simulink model "s_b16a4x512f"  (R2016b)
settings: Solver=VariableStepDiscrete  StartTime=0.0  StopTime=1  RelTol=1e-3
undefined symbols (not defined in the file): fft_stages, n_bits_ants, n_bits_xengs
libraries: xbsIndex_r4 x23057, casper_library_misc x150, xbsReplacements_r4 x9, casper_library_delays x8, xps_library x3
(part 59 of 210)

== system s_b16a4x512f/sys2/pack_out_skarab/pack_xeng ==
  note: eof ON the last valid data.
  note: SPEAD header
  note: magic number - 0x53
  note: spead version
  note: item id width in bytes
  note: heap addr width in bytes
  note: <reserved>
  note: num item pointers -
      | after this header
  data256_ready : Inport
  data256_valid : Inport  Port=2
  data256 : Inport  Port=3
  hdr_heap_id : Inport  Port=4
  hdr_heap_size : Inport  Port=5
  hdr_heap_offset : Inport  Port=6
  hdr_pkt_len_words : Inport  Port=7
  hdr5_0x1600_DIR : Inport  Port=8
  hdr6_0x4103_DIR : Inport  Port=9
  hdr8_0x1800 : Inport  Port=10
  AddSub1 : xbsIndex_r4/AddSub  mode=Subtraction  use_carryin=off  use_carryout=off  en=off  latency=0  precision=Full  arith_type=Unsigned  n_bits=16  bin_pt=14  quantization=Truncate  overflow=Wrap  use_behavioral_HDL=off  hw_selection=Fabric  pipelined=off  dbl_ovrd=off  block_type=addsub
  Assert17 : xbsIndex_r4/Assert  assert_type=on  type_source=Explicitly  gui_display_data_type=Fixed-point  arith_type=Unsigned  n_bits=64  bin_pt=0  preci_type=Single  exp_width=8  frac_width=24  assert_rate=off  rate_source=Explicitly  period=1  output_port=on  block_type=assert
  Assert18 : xbsIndex_r4/Assert  assert_type=on  type_source=Explicitly  gui_display_data_type=Fixed-point  arith_type=Unsigned  n_bits=256  bin_pt=0  preci_type=Single  exp_width=8  frac_width=24  assert_rate=off  rate_source=Explicitly  period=1  output_port=on  block_type=assert
  Assert5 : xbsIndex_r4/Assert  assert_type=on  type_source=Explicitly  gui_display_data_type=Fixed-point  arith_type=Boolean  n_bits=64  bin_pt=0  preci_type=Single  exp_width=8  frac_width=24  assert_rate=off  rate_source=Explicitly  period=1  output_port=on  block_type=assert
      settings: block_version=10.1.3
  Assert6 : xbsIndex_r4/Assert  assert_type=on  type_source=Explicitly  gui_display_data_type=Fixed-point  arith_type=Unsigned  n_bits=256  bin_pt=0  preci_type=Single  exp_width=8  frac_width=24  assert_rate=off  rate_source=Explicitly  period=1  output_port=on  block_type=assert
      settings: block_version=10.1.3
  Assert7 : xbsIndex_r4/Assert  assert_type=on  type_source=Explicitly  gui_display_data_type=Boolean  arith_type=Boolean  n_bits=64  bin_pt=0  preci_type=Single  exp_width=8  frac_width=24  assert_rate=off  rate_source=Explicitly  period=1  output_port=on  block_type=assert
      settings: block_version=10.1.3
  Concat : xbsIndex_r4/Concat  num_inputs=6  dbl_ovrd=off  block_type=concat
      settings: block_version=10.1.3
  Concat1 : xbsIndex_r4/Concat  num_inputs=4  dbl_ovrd=off  block_type=concat
      settings: block_version=10.1.3
  Concat3 : xbsIndex_r4/Concat  num_inputs=4  dbl_ovrd=off  block_type=concat
      settings: block_version=10.1.3
  Constant3 : xbsIndex_r4/Constant  const=83  gui_display_data_type=Fixed-point  arith_type=Unsigned  n_bits=8  bin_pt=0  preci_type=Single  exp_width=8  frac_width=24  explicit_period=on  period=1  equ=P=C  opselect=C  inp2=PCIN>>17  opr=+  inp1=P  carry=CIN  dbl_ovrd=off  block_type=constant
  Constant4 : xbsIndex_r4/Constant  const=spead_version  gui_display_data_type=Fixed-point  arith_type=Unsigned  n_bits=8  bin_pt=0  preci_type=Single  exp_width=8  frac_width=24  explicit_period=on  period=1  equ=P=C  opselect=C  inp2=PCIN>>17  opr=+  inp1=P  carry=CIN  dbl_ovrd=off  block_type=constant
  Constant7 : xbsIndex_r4/Constant  const=0  gui_display_data_type=Fixed-point  arith_type=Unsigned  n_bits=16  bin_pt=0  preci_type=Single  exp_width=8  frac_width=24  explicit_period=on  period=1  equ=P=C  opselect=C  inp2=PCIN>>17  opr=+  inp1=P  carry=CIN  dbl_ovrd=off  block_type=constant
  Logical5 : xbsIndex_r4/Logical  logical_function=AND  inputs=2  en=off  latency=0  precision=Full  arith_type=Unsigned  n_bits=8  bin_pt=2  align_bp=on  dbl_ovrd=off  block_type=logical
      settings: xl_area=[0, 0, 0, 0, 0, 0, 0]
  Logical6 : xbsIndex_r4/Logical  logical_function=OR  inputs=2  en=off  latency=0  precision=Full  arith_type=Unsigned  n_bits=8  bin_pt=2  align_bp=on  dbl_ovrd=off  block_type=logical
      settings: xl_area=[0, 0, 0, 0, 0, 0, 0]
  Logical7 : xbsIndex_r4/Logical  logical_function=OR  inputs=2  en=off  latency=1  precision=Full  arith_type=Unsigned  n_bits=8  bin_pt=2  align_bp=on  dbl_ovrd=off  block_type=logical
      settings: xl_area=[0, 0, 0, 0, 0, 0, 0]
  Logical8 : xbsIndex_r4/Logical  logical_function=OR  inputs=2  en=off  latency=0  precision=Full  arith_type=Unsigned  n_bits=8  bin_pt=2  align_bp=on  dbl_ovrd=off  block_type=logical
      settings: xl_area=[0, 0, 0, 0, 0, 0, 0]
  Register2 : xbsIndex_r4/Register  init=0  rst=on  en=on  dbl_ovrd=off  block_type=register
  Relational3 : xbsIndex_r4/Relational  mode=a=b  op_type=Bool  en=off  latency=0  dbl_ovrd=off  block_type=relational
      settings: xl_area=[0, 0, 0, 0, 0, 0, 0]  block_version=10.1.3
  assert_data2 : xbsIndex_r4/Assert  assert_type=on  type_source=Explicitly  gui_display_data_type=Fixed-point  arith_type=Unsigned  n_bits=256  bin_pt=0  preci_type=Single  exp_width=8  frac_width=24  assert_rate=off  rate_source=Explicitly  period=1  output_port=on  block_type=assert
  assert_data3 : xbsIndex_r4/Assert  assert_type=on  type_source=Explicitly  gui_display_data_type=Fixed-point  arith_type=Unsigned  n_bits=256  bin_pt=0  preci_type=Single  exp_width=8  frac_width=24  assert_rate=off  rate_source=Explicitly  period=1  output_port=on  block_type=assert
  data_ctr1 : xbsIndex_r4/Counter  cnt_type=Free Running  cnt_to=4  operation=Up  start_count=0  cnt_by_val=1  arith_type=Unsigned  n_bits=max_pkt_len_bits + 1  bin_pt=0  load_pin=off  rst=on  en=on  explicit_period=on  period=1  use_behavioral_HDL=off  implementation=Fabric  use_rpm=on  dbl_ovrd=off  block_type=counter
      settings: xl_area=[0, 0, 0, 0, 0, 0, 0]
  delay_data{6,9..10,13,15,17..18,20} (8 alike) : xbsIndex_r4/Delay  rst=off  infoeditControl=Selection of Reset will increase slice count due to use of real FFs and instead of SRLs  en=off  latency=1  reg_retiming=on  dbl_ovrd=off  block_type=delay
      settings: block_version=11.4
  delay_data12 : xbsIndex_r4/Delay  rst=off  infoeditControl=Selection of Reset will increase slice count due to use of real FFs and instead of SRLs  en=off  latency=2  reg_retiming=on  dbl_ovrd=off  block_type=delay
      settings: infoedit=Hardware notes: A delay line is a chain, each link of which is an SRL16 or SRL32 followed by a flip-flop.  block_version=11.4
  delay_data5 : xbsIndex_r4/Delay  rst=off  infoeditControl=Selection of Reset will increase slice count due to use of real FFs and instead of SRLs  en=off  latency=2  reg_retiming=on  dbl_ovrd=off  block_type=delay
      settings: infoedit=Hardware notes: A delay line is a chain, each link of which is an SRL16 or SRL32 followed by a flip-flop.  block_version=11.4
  delay_data7 : xbsIndex_r4/Delay  rst=off  infoeditControl=Selection of Reset will increase slice count due to use of real FFs and instead of SRLs  en=off  latency=2  reg_retiming=on  dbl_ovrd=off  block_type=delay
      settings: infoedit=Hardware notes: A delay line is a chain, each link of which is an SRL16 or SRL32 followed by a flip-flop.  block_version=11.4
  hdra_{1..6,8} (7 alike) : xbsIndex_r4/Assert  assert_type=on  type_source=Explicitly  gui_display_data_type=Fixed-point  arith_type=Unsigned  n_bits=spead_lsw  bin_pt=0  preci_type=Single  exp_width=8  frac_width=24  assert_rate=off  rate_source=Explicitly  period=1  output_port=on  block_type=assert
  header_4cast4 : xbsIndex_r4/Convert  gui_display_data_type=Fixed-point  arith_type=Unsigned  n_bits=spead_lsw - 5  bin_pt=0  float_type=Single  exp_bits=8  fraction_bits=24  quantization=Truncate  overflow=Wrap  en=off  latency=1  pipeline=on  dbl_ovrd=off  block_type=convert
  header_4cat4 : xbsIndex_r4/Concat  num_inputs=2  dbl_ovrd=off  block_type=concat
  header_4const2 : xbsIndex_r4/Constant  const=0  gui_display_data_type=Fixed-point  arith_type=Unsigned  n_bits=spead_lsw  bin_pt=0  preci_type=Single  exp_width=8  frac_width=24  explicit_period=on  period=1  equ=P=C  opselect=C  inp2=PCIN>>17  opr=+  inp1=P  carry=CIN  dbl_ovrd=off  block_type=constant
  header_4const4 : xbsIndex_r4/Constant  const=0  gui_display_data_type=Fixed-point  arith_type=Unsigned  n_bits=5  bin_pt=0  preci_type=Single  exp_width=8  frac_width=24  explicit_period=on  period=1  equ=P=C  opselect=C  inp2=PCIN>>17  opr=+  inp1=P  carry=CIN  dbl_ovrd=off  block_type=constant
  header_assert{1..6,8} (7 alike) : xbsIndex_r4/Assert  assert_type=on  type_source=Explicitly  gui_display_data_type=Fixed-point  arith_type=Unsigned  n_bits=spead_msw  bin_pt=0  preci_type=Single  exp_width=8  frac_width=24  assert_rate=off  rate_source=Explicitly  period=1  output_port=on  block_type=assert
  header_cat{1..6,8} (7 alike) : xbsIndex_r4/Concat  num_inputs=2  dbl_ovrd=off  block_type=concat
  header_const1 : xbsIndex_r4/Constant  const=32769  gui_display_data_type=Fixed-point  arith_type=Unsigned  n_bits=spead_msw - spead_lsw  bin_pt=0  preci_type=Single  exp_width=8  frac_width=24  explicit_period=off  period=1  equ=P=C  opselect=C  inp2=PCIN>>17  opr=+  inp1=P  carry=CIN  dbl_ovrd=off  block_type=constant
  header_const2 : xbsIndex_r4/Constant  const=32770  gui_display_data_type=Fixed-point  arith_type=Unsigned  n_bits=spead_msw - spead_lsw  bin_pt=0  preci_type=Single  exp_width=8  frac_width=24  explicit_period=off  period=1  equ=P=C  opselect=C  inp2=PCIN>>17  opr=+  inp1=P  carry=CIN  dbl_ovrd=off  block_type=constant
  header_const3 : xbsIndex_r4/Constant  const=32771  gui_display_data_type=Fixed-point  arith_type=Unsigned  n_bits=spead_msw - spead_lsw  bin_pt=0  preci_type=Single  exp_width=8  frac_width=24  explicit_period=off  period=1  equ=P=C  opselect=C  inp2=PCIN>>17  opr=+  inp1=P  carry=CIN  dbl_ovrd=off  block_type=constant
  header_const4 : xbsIndex_r4/Constant  const=32772  gui_display_data_type=Fixed-point  arith_type=Unsigned  n_bits=spead_msw - spead_lsw  bin_pt=0  preci_type=Single  exp_width=8  frac_width=24  explicit_period=off  period=1  equ=P=C  opselect=C  inp2=PCIN>>17  opr=+  inp1=P  carry=CIN  dbl_ovrd=off  block_type=constant
  header_const5 : xbsIndex_r4/Constant  const=38400  gui_display_data_type=Fixed-point  arith_type=Unsigned  n_bits=spead_msw - spead_lsw  bin_pt=0  preci_type=Single  exp_width=8  frac_width=24  explicit_period=off  period=1  equ=P=C  opselect=C  inp2=PCIN>>17  opr=+  inp1=P  carry=CIN  dbl_ovrd=off  block_type=constant
  header_const6 : xbsIndex_r4/Constant  const=49411  gui_display_data_type=Fixed-point  arith_type=Unsigned  n_bits=spead_msw - spead_lsw  bin_pt=0  preci_type=Single  exp_width=8  frac_width=24  explicit_period=off  period=1  equ=P=C  opselect=C  inp2=PCIN>>17  opr=+  inp1=P  carry=CIN  dbl_ovrd=off  block_type=constant
  header_const8 : xbsIndex_r4/Constant  const=6144  gui_display_data_type=Fixed-point  arith_type=Unsigned  n_bits=spead_msw - spead_lsw  bin_pt=0  preci_type=Single  exp_width=8  frac_width=24  explicit_period=off  period=1  equ=P=C  opselect=C  inp2=PCIN>>17  opr=+  inp1=P  carry=CIN  dbl_ovrd=off  block_type=constant
  heap_addr_width : xbsIndex_r4/Constant  const=spead_lsw/8  gui_display_data_type=Fixed-point  arith_type=Unsigned  n_bits=8  bin_pt=0  preci_type=Single  exp_width=8  frac_width=24  explicit_period=on  period=1  equ=P=C  opselect=C  inp2=PCIN>>17  opr=+  inp1=P  carry=CIN  dbl_ovrd=off  block_type=constant
  item_id_width : xbsIndex_r4/Constant  const=(spead_msw-spead_lsw)/8  gui_display_data_type=Fixed-point  arith_type=Unsigned  n_bits=8  bin_pt=0  preci_type=Single  exp_width=8  frac_width=24  explicit_period=on  period=1  equ=P=C  opselect=C  inp2=PCIN>>17  opr=+  inp1=P  carry=CIN  dbl_ovrd=off  block_type=constant
  mainmux1 : xbsIndex_r4/Mux  inputs=2  en=off  latency=1  precision=Full  arith_type="Signed  (2's comp)"  n_bits=8  bin_pt=2  quantization=Truncate  overflow=Wrap  dbl_ovrd=off  block_type=mux
      settings: xl_area=[0, 0, 0, 0, 0, 0, 0]
  mainmux2 : xbsIndex_r4/Mux  inputs=2  en=off  latency=1  precision=Full  arith_type="Signed  (2's comp)"  n_bits=8  bin_pt=2  quantization=Truncate  overflow=Wrap  dbl_ovrd=off  block_type=mux
      settings: xl_area=[0, 0, 0, 0, 0, 0, 0]
  num_item_pts : xbsIndex_r4/Constant  const=7  gui_display_data_type=Fixed-point  arith_type=Unsigned  n_bits=16  bin_pt=0  preci_type=Single  exp_width=8  frac_width=24  explicit_period=on  period=1  equ=P=C  opselect=C  inp2=PCIN>>17  opr=+  inp1=P  carry=CIN  dbl_ovrd=off  block_type=constant
  only_one1 : xbsIndex_r4/Constant  const=1  gui_display_data_type=Fixed-point  arith_type=Unsigned  n_bits=1  bin_pt=0  preci_type=Single  exp_width=8  frac_width=24  explicit_period=on  period=1  equ=P=C  opselect=C  inp2=PCIN>>17  opr=+  inp1=P  carry=CIN  dbl_ovrd=off  block_type=constant
  data_out : Outport
  valid_out : Outport  Port=2
  eof : Outport  Port=3
  data_overflow : Outport  Port=4
  wires:
  [out_data] -> Assert18/1
  [out_valid] -> valid_out/1
  [out_overflow] -> data_overflow/1
  [out_done] -> eof/1
  Logical8/1 -> [out_done]  "out_done"
  delay_data20/1 -> [out_overflow], Logical8/2  "out_overflow"
  delay_data18/1 -> delay_data20/1
  Logical5/1 -> delay_data18/1  "overflow"
  Register2/1 -> Logical5/1  "busy"
  delay_data17/1 -> Logical8/1
  delay_data15/1 -> delay_data17/1
  Relational3/1 -> delay_data15/1, Register2/2  "done"
  AddSub1/1 -> Relational3/2
  only_one1/1 -> AddSub1/2
  [hdr_4] -> AddSub1/1
  data_ctr1/1 -> Relational3/1  "data_ctr"
  [in_data256] -> delay_data12/1
  delay_data12/1 -> delay_data13/1
  delay_data9/1 -> [out_valid]  "out_valid"
  Logical7/1 -> delay_data9/1
  [header1] -> mainmux2/3
  [header0] -> mainmux2/2
  delay_data7/1 -> Logical6/2, mainmux2/1
  mainmux1/1 -> [out_data]  "out_data"
  delay_data13/1 -> mainmux1/2
  mainmux2/1 -> mainmux1/3
  delay_data10/1 -> mainmux1/1
  delay_data6/1 -> Logical6/1
  Logical6/1 -> Logical7/1, data_ctr1/1, delay_data10/1  "wr_hdr"
  [in_ready] -> delay_data6/1, delay_data7/1, Register2/1, Register2/3, Logical5/2  "in_rdy"
  delay_data5/1 -> Logical7/2, data_ctr1/2  "wr_data"
  [in_valid] -> delay_data5/1
  assert_data3/1 -> [header1]
  Concat3/1 -> assert_data3/1
  assert_data2/1 -> [header0]
  Concat1/1 -> assert_data2/1
  header_cat8/1 -> header_assert8/1
  [hdr_8] -> header_cat8/2
  header_const8/1 -> header_cat8/1  "spid8"
  hdra_8/1 -> [hdr_8]  "hdr8_0x4300"
  hdr8_0x1800/1 -> hdra_8/1
  header_assert8/1 -> Concat3/4
  header_assert6/1 -> Concat3/3
  header_cat6/1 -> header_assert6/1
  [hdr_6] -> header_cat6/2
  header_const6/1 -> header_cat6/1  "spid6"
  hdra_6/1 -> [hdr_6]  "hdr6_0x4101_DIR"
  hdr6_0x4103_DIR/1 -> hdra_6/1
  header_assert5/1 -> Concat3/2
  header_cat5/1 -> header_assert5/1
  [hdr_5] -> header_cat5/2
  header_const5/1 -> header_cat5/1  "spid5"
  hdra_5/1 -> [hdr_5]  "hdr5_0x1600_DIR"
  hdr5_0x1600_DIR/1 -> hdra_5/1
  header_assert4/1 -> Concat3/1
  header_cat4/1 -> header_assert4/1
  header_4cat4/1 -> header_cat4/2
  header_4const4/1 -> header_4cat4/2
  header_4cast4/1 -> header_4cat4/1
  [hdr_4] -> header_4cast4/1
  header_const4/1 -> header_cat4/1  "spid4"
  hdra_4/1 -> [hdr_4]  "hdr_pkt_len_words"
  hdr_pkt_len_words/1 -> hdra_4/1
  header_assert3/1 -> Concat1/4
  header_cat3/1 -> header_assert3/1
  [hdr_3] -> header_cat3/2
  header_const3/1 -> header_cat3/1  "spid3"
  hdra_3/1 -> [hdr_3]  "hdr_heap_offset"
  hdr_heap_offset/1 -> hdra_3/1
  header_assert2/1 -> Concat1/3
  header_cat2/1 -> header_assert2/1
  [hdr_2] -> header_cat2/2
  header_const2/1 -> header_cat2/1  "spid2"
  hdra_2/1 -> [hdr_2]  "hdr_heap_size"
  hdr_heap_size/1 -> hdra_2/1
  header_assert1/1 -> Concat1/2
  header_cat1/1 -> header_assert1/1
  [hdr_1] -> header_cat1/2
  header_const1/1 -> header_cat1/1  "spid1"
  hdra_1/1 -> [hdr_1]  "hdr_heap_id"
  hdr_heap_id/1 -> hdra_1/1
  num_item_pts/1 -> Concat/6
  Assert18/1 -> data_out/1
  Assert17/1 -> Concat1/1
  Assert7/1 -> [in_valid]  "data64_valid"
  data256_valid/1 -> Assert7/1
  data256_ready/1 -> Assert5/1
  Assert5/1 -> [in_ready]  "data64_rdy"
  Assert6/1 -> [in_data256]  "data64"
  data256/1 -> Assert6/1
  Constant7/1 -> Concat/5
  heap_addr_width/1 -> Concat/4
  item_id_width/1 -> Concat/3
  Constant4/1 -> Concat/2
  Constant3/1 -> Concat/1
  Concat/1 -> Assert17/1  "spd_hdr"

== system s_b16a4x512f/sys2/pkt_reord/bus_expand ==
  bus_in : Inport
  reinterpret1 : xbsIndex_r4/Reinterpret  force_arith_type=on  arith_type=Unsigned  force_bin_pt=on  bin_pt=0  block_type=reinterpret
  slice1 : xbsIndex_r4/Slice  nbits=32  boolean_output=off  mode=Upper Bit Location + Width  bit1=-1  base1=MSB of Input  bit0=0  base0=LSB of Input  dbl_ovrd=off  block_type=slice
  slice2 : xbsIndex_r4/Slice  nbits=1  boolean_output=on  mode=Upper Bit Location + Width  bit1=0  base1=MSB of Input  bit0=0  base0=LSB of Input  dbl_ovrd=off  block_type=slice
  msb_out2 : Outport
  lsb_out1 : Outport  Port=2
  wires:
  bus_in/1 -> slice2/1, slice1/1
  slice2/1 -> msb_out2/1
  slice1/1 -> reinterpret1/1
  reinterpret1/1 -> lsb_out1/1

== system s_b16a4x512f/sys2/pkt_reord/bus_replicate ==
  in : Inport
  bussify : Subsystem  AncestorBlock=casper_library_flow_control/bus_create  mask(bus_create){inputNum=1}
      mask prompts: inputNum "Number of inputs:"
      mask init:
      | bus_create_init(gcb,...
      |     'inputNum', inputNum);
  out : Outport
  wires:
  in/1 -> bussify/1(in1)
  bussify/1(bus_out) -> out/1

== system s_b16a4x512f/sys2/pkt_reord/input_control ==
  note: signal discard if timestamp
      | changing i.e new packet
      | and not writing
      | and valid
  note: Allow writing to windows
      | up to 1/2 the total buffer size
      |  behind the current maximum
      | mcnt
  data_in : Inport
  valid : Inport  Port=2
  pkt_idx : Inport  Port=3
  time_freq : Inport  Port=4
  src : Inport  Port=5
  pkt_size : Inport  Port=6
  n_src : Inport  Port=7
  AddSub2 : xbsIndex_r4/AddSub  mode=Addition  use_carryin=off  use_carryout=off  en=off  latency=2  precision=User Defined  arith_type=Unsigned  n_bits=n_bits_timestamp+chan_bits-xeng_bits  bin_pt=0  quantization=Truncate  overflow=Wrap  use_behavioral_HDL=on  hw_selection=Fabric  pipelined=off  use_rpm=on  dbl_ovrd=off  block_type=addsub
      settings: xl_area=[0, 0, 0, 0, 0, 0, 0]  block_version=10.1.3
  Constant2 : xbsIndex_r4/Constant  const=2^(window_bits - 1)  gui_display_data_type=Fixed-point  arith_type=Unsigned  n_bits=n_bits_timestamp+chan_bits-xeng_bits  bin_pt=0  preci_type=Single  exp_width=8  frac_width=24  explicit_period=on  period=1  equ=P=C  opselect=C  inp2=PCIN>>17  opr=+  inp1=P  carry=CIN  dbl_ovrd=off  block_type=constant
  Constant4 : xbsIndex_r4/Constant  const=0  gui_display_data_type=Boolean  arith_type=Boolean  n_bits=16  bin_pt=14  preci_type=Single  exp_width=8  frac_width=24  explicit_period=on  period=1  equ=P=C  opselect=C  inp2=PCIN>>17  opr=+  inp1=P  carry=CIN  dbl_ovrd=off  block_type=constant
      settings: block_version=11.4
  Delay{6,11,13..16} (6 alike) : xbsIndex_r4/Delay  rst=off  infoeditControl=Selection of Reset will increase slice count due to use of real FFs and instead of SRLs  en=off  latency=1  reg_retiming=on  dbl_ovrd=off  block_type=delay
      Delay11 settings: infoedit=Hardware notes: A delay line is a chain, each link of which is an SRL16 or SRL32 followed by a flip-flop.  xl_area=[0, 0, 0, 0, 0, 0, 0]
      Delay13 settings: infoedit=Hardware notes: A delay line is a chain, each link of which is an SRL16 or SRL32 followed by a flip-flop.  xl_area=[0, 0, 0, 0, 0, 0, 0]
      Delay14 settings: infoedit=Hardware notes: A delay line is a chain, each link of which is an SRL16 or SRL32 followed by a flip-flop.  xl_area=[0, 0, 0, 0, 0, 0, 0]
      Delay15 settings: infoedit=Hardware notes: A delay line is a chain, each link of which is an SRL16 or SRL32 followed by a flip-flop.  xl_area=[0, 0, 0, 0, 0, 0, 0]
      Delay16 settings: infoedit=Hardware notes: A delay line is a chain, each link of which is an SRL16 or SRL32 followed by a flip-flop.  xl_area=[0, 0, 0, 0, 0, 0, 0]
      Delay6 settings: xl_area=[0, 0, 0, 0, 0, 0, 0]
  Delay{2,4..5,8..9} (5 alike) : xbsIndex_r4/Delay  rst=off  infoeditControl=Selection of Reset will increase slice count due to use of real FFs and instead of SRLs  en=off  latency=2  reg_retiming=on  dbl_ovrd=off  block_type=delay
      settings: xl_area=[0, 0, 0, 0, 0, 0, 0]
  Delay{3,21,24..27} (6 alike) : xbsIndex_r4/Delay  rst=off  infoeditControl=Selection of Reset will increase slice count due to use of real FFs and instead of SRLs  en=off  latency=3  reg_retiming=on  dbl_ovrd=off  block_type=delay
      settings: xl_area=[0, 0, 0, 0, 0, 0, 0]
  Delay23 : xbsIndex_r4/Delay  rst=off  infoeditControl=Selection of Reset will increase slice count due to use of real FFs and instead of SRLs  en=off  latency=4  reg_retiming=on  dbl_ovrd=off  block_type=delay
      settings: xl_area=[0, 0, 0, 0, 0, 0, 0]
  Gateway Out{1..19} (19 alike) : xbsIndex_r4/Gateway Out  inherit_from_input=off  hdl_port=off  rows=1  columns=1  UseAsDAC=off  DACChannel='1'  interface=None  automatic_assignment=on  address_offset=hex2dec('00')  intf_name=''  intf_description=''  timing_constraint=None  locs_specified=off  LOCs={}  io_standard={}  block_type=gatewayout
      settings: infoedit="Gateway out block.  Converts Xilinx fixed point inputs into ouputs of type Simulink integer, double, or fixed point.<P><P>Hardware notes:  In hardware these blocks become top level output ports or are discarded, depending on how they are configured."  xl_area=[0, 0, 0, 0, 0, 0, 0]  block_version=10.1.3
  Inverter : xbsIndex_r4/Inverter  en=off  latency=0  dbl_ovrd=off  block_type=inv
  Logical : xbsIndex_r4/Logical  logical_function=AND  inputs=3  en=off  latency=1  precision=Full  arith_type=Unsigned  n_bits=8  bin_pt=2  align_bp=on  dbl_ovrd=off  block_type=logical
      settings: xl_area=[0, 0, 0, 0, 0, 0, 0]
  Logical1 : xbsIndex_r4/Logical  logical_function=AND  inputs=3  en=off  latency=0  precision=Full  arith_type=Unsigned  n_bits=8  bin_pt=2  align_bp=on  dbl_ovrd=off  block_type=logical
      settings: xl_area=[0, 0, 0, 0, 0, 0, 0]
  Mult : xbsIndex_r4/Mult  precision=Full  arith_type=Unsigned  n_bits=buf_bits  bin_pt=0  quantization=Truncate  overflow=Wrap  en=off  latency=3  use_behavioral_HDL=off  opt=Speed  use_embedded=on  optimum_pipeline=off  pipeline=on  dbl_ovrd=off  use_rpm=on  placement_style=Triangular  block_type=mult
  Mult1 : xbsIndex_r4/Mult  precision=Full  arith_type=Unsigned  n_bits=buf_bits  bin_pt=0  quantization=Truncate  overflow=Wrap  en=off  latency=3  use_behavioral_HDL=off  opt=Speed  use_embedded=on  optimum_pipeline=off  pipeline=on  dbl_ovrd=off  use_rpm=on  placement_style=Triangular  block_type=mult
  Relational : xbsIndex_r4/Relational  mode=a>=b  op_type=Bool  en=off  latency=2  dbl_ovrd=off  block_type=relational
      settings: xl_area=[0, 0, 0, 0, 0, 0, 0]  block_version=10.1.3
  Relational1 : xbsIndex_r4/Relational  mode=a!=b  op_type=Bool  en=off  latency=2  dbl_ovrd=off  block_type=relational
  Relational2 : xbsIndex_r4/Relational  mode=a<b  op_type=Bool  en=off  latency=2  dbl_ovrd=off  block_type=relational
      settings: xl_area=[0, 0, 0, 0, 0, 0, 0]  block_version=10.1.3
  Scope : Scope  NumInputPorts=7
  Slice1 : xbsIndex_r4/Slice  nbits=buf_bits  boolean_output=off  mode=Lower Bit Location + Width  bit1=0  base1=MSB of Input  bit0=0  base0=LSB of Input  dbl_ovrd=off  block_type=slice
  Slice2 : xbsIndex_r4/Slice  nbits=window_bits  boolean_output=off  mode=Lower Bit Location + Width  bit1=0  base1=MSB of Input  bit0=0  base0=LSB of Input  dbl_ovrd=off  block_type=slice
  Slice5 : xbsIndex_r4/Slice  nbits=8  boolean_output=off  mode=Lower Bit Location + Width  bit1=0  base1=MSB of Input  bit0=0  base0=LSB of Input  dbl_ovrd=off  block_type=slice
  Terminator : Terminator
  adder_tree : Subsystem  AncestorBlock=casper_library_misc/adder_tree  mask(adder_tree){n_inputs=3, latency=2, adder_imp=Fabric, first_stage_hdl=off}
      mask prompts: n_inputs "Number of Inputs"; latency "Add Latency"; adder_imp "Adder implementation"; first_stage_hdl "Use behavioural HDL for first stage of adders"
      mask help:
      | Sums all inputs using a tree of adds and delays.
      |
      | Number of inputs: The number of inputs to the block to be summed
      | Add latency: The number of clock cycles to perform one addition (affects timing)..
      | Adder implementation: choice of fabric or DSP48E core, or behavioral HDL
      | Use behavioural HDL for first stage of adders: Causes the first stage of adders to be absorbed into DSP blocks if multipliers precede them (Virtex 5). Overrides Adder implementation
      mask init:
      | adder_tree_init(gcb, ...
      |     'n_inputs', n_inputs, ...
      |     'latency', latency, ...
      |     'adder_imp', adder_imp, ...
      |     'first_stage_hdl', first_stage_hdl);
      settings: AttributesFormatString=latency 4
      mask Help: eval('xlWeb(''http://casper.berkeley.edu/wiki/Adder_tree'')')
      mask TypeOptions adder_imp: Behavioral | Fabric | DSP48
  freq_window : xbsIndex_r4/Mult  precision=Full  arith_type="Signed  (2's comp)"  n_bits=16  bin_pt=14  quantization=Truncate  overflow=Wrap  en=off  latency=3  use_behavioral_HDL=off  opt=Speed  use_embedded=on  optimum_pipeline=off  pipeline=on  dbl_ovrd=off  use_rpm=on  placement_style=Triangular  block_type=mult
  internal_descr_Scope2 : Scope  NumInputPorts=6
  internal_descr_Scope3 : Scope  NumInputPorts=6
  mcnt_thresh : Subsystem
  maxcnt : Outport
  wr_addr : Outport  Port=2
  wr_data : Outport  Port=3
  we : Outport  Port=4
  discarding : Outport  Port=5
  mcnt_timeout : Outport  Port=6
  wires:
  Constant2/1 -> AddSub2/2
  Delay2/1 -> Delay4/1
  Delay3/1 -> Delay2/1, [data_add]
  data_in/1 -> Delay3/1
  adder_tree/2(dout) -> Slice1/1
  Gateway Out15/1 -> internal_descr_Scope3/6
  [brds_pkt_size_time] -> Gateway Out15/1
  [src_pkt_size] -> Gateway Out9/1
  Slice5/1 -> Gateway Out6/1
  Gateway Out1/1 -> internal_descr_Scope3/2
  Gateway Out6/1 -> internal_descr_Scope3/1
  Gateway Out7/1 -> internal_descr_Scope3/3
  Gateway Out9/1 -> internal_descr_Scope3/4
  Gateway Out14/1 -> internal_descr_Scope3/5
  [data_add] -> Slice5/1
  [valid_add] -> Gateway Out1/1
  [pkt_idx] -> Gateway Out7/1
  [wr_addr] -> Gateway Out14/1
  [wr_data] -> Gateway Out3/1
  Gateway Out2/1 -> internal_descr_Scope2/2
  Gateway Out3/1 -> internal_descr_Scope2/1
  Gateway Out4/1 -> internal_descr_Scope2/3
  Gateway Out5/1 -> internal_descr_Scope2/4
  Gateway Out16/1 -> internal_descr_Scope2/5
  [we] -> Gateway Out2/1
  [mcnt_in] -> Gateway Out4/1
  [max_mcnt] -> Gateway Out5/1
  [wr_addr] -> Gateway Out16/1
  Slice2/1 -> Mult1/2
  freq_window/1 -> Mult1/1
  n_src/1 -> freq_window/1
  Mult1/1 -> adder_tree/2(din1), [brds_pkt_size_time]
  Delay27/1 -> AddSub2/1
  Delay26/1 -> mcnt_thresh/1(mcnt)
  Delay25/1 -> Delay5/1
  Constant4/1 -> adder_tree/1(sync)
  Mult/1 -> adder_tree/3(din2), [src_pkt_size]
  Delay21/1 -> [pkt_idx], adder_tree/4(din3)
  time_freq/1 -> Slice2/1, Delay26/1, Delay25/1, [mcnt_in], Delay27/1
  Delay24/1 -> mcnt_thresh/2(en), [valid_add], Delay23/1
  src/1 -> Mult/1
  pkt_size/1 -> freq_window/2, Mult/2
  pkt_idx/1 -> Delay21/1
  valid/1 -> Delay24/1
  Delay9/1 -> Delay13/1
  Slice1/1 -> Delay16/1
  Delay4/1 -> Delay11/1
  Delay23/1 -> Gateway Out13/1, Logical/3, Delay14/1
  Logical/1 -> [we], Inverter/1, we/1
  Relational/1 -> Gateway Out12/1, Logical/2
  Delay5/1 -> Gateway Out10/1, Relational/2, Relational1/1, Delay6/1
  mcnt_thresh/1(maxcnt) -> Delay9/1, Relational2/1, Relational/1, Gateway Out19/1
  Relational2/1 -> Logical/1, Gateway Out11/1
  adder_tree/1(sync_out) -> Terminator/1
  Logical1/1 -> [discarding], discarding/1
  Inverter/1 -> Logical1/1
  Relational1/1 -> Delay15/1, Gateway Out17/1
  Delay6/1 -> Relational1/2
  mcnt_thresh/2(mcnt_timeout) -> Delay8/1
  [discarding] -> Gateway Out8/1
  Gateway Out8/1 -> internal_descr_Scope2/6
  Gateway Out11/1 -> Scope/4
  Gateway Out18/1 -> Scope/3
  Gateway Out13/1 -> Scope/6
  Gateway Out17/1 -> Scope/7
  Gateway Out12/1 -> Scope/5
  Gateway Out10/1 -> Scope/1
  Gateway Out19/1 -> Scope/2
  AddSub2/1 -> Gateway Out18/1, Relational2/2
  Delay11/1 -> wr_data/1, [wr_data]
  Delay13/1 -> maxcnt/1, [max_mcnt]
  Delay14/1 -> Logical1/2
  Delay15/1 -> Logical1/3
  Delay8/1 -> mcnt_timeout/1
  Delay16/1 -> [wr_addr], wr_addr/1

== system s_b16a4x512f/sys2/pkt_reord/munge ==
  din : Inport
  join : Subsystem  AncestorBlock=casper_library_flow_control/bus_create  mask(bus_create){inputNum=16}
      mask prompts: inputNum "Number of inputs:"
      mask init:
      | bus_create_init(gcb,...
      |     'inputNum', inputNum);
  reinterpret : xbsIndex_r4/Reinterpret  force_arith_type=on  arith_type=Unsigned  force_bin_pt=on  bin_pt=0  block_type=reinterpret
  reinterpret_out : xbsIndex_r4/Reinterpret  force_arith_type=on  arith_type=Unsigned  force_bin_pt=on  bin_pt=0  block_type=reinterpret
  split : Subsystem  AncestorBlock=casper_library_flow_control/bus_expand  mask(bus_expand){mode=divisions of arbitrary size, outputNum=1, outputWidth=[1 32 32 32 32 32 32 32 32], outputBinaryPt=[0 0 0 0 0 0 0 0 0], outputArithmeticType=[0 0 0 0 0 0 0 0 0], show_format=off, outputToWorkspace=off, variablePrefix=out, outputToModelAsWell=on}
      mask prompts: outputNum "Number of outputs:"; outputWidth "Output width [msb ... lsb]:"; outputBinaryPt "Output binary point position [msb ... lsb]:"; outputArithmeticType "Output arithmetic type (ufix=0, fix=1, bool=2) [msb ... lsb]:"; show_format "Print format string?"; outputToWorkspace "Output to workspace?"; variablePrefix "Variable name prefix:"; outputToModelAsWell "Output to model as well?"
      mask help:
      | Expands a 'bus' made using a bus_create or Xilinx
      | concat block.
      | The input will be divided into the specified number
      | of outputs with the specified arithmetic types.
      | Divisions are made from most significant bit.
      mask init: same as s_b16a4x512f/bus_expand
      settings: AttributesFormatString=9 outputs
      mask TypeOptions mode: divisions of equal size | divisions of arbitrary size
      mask Callback mode: bus_expand_callback();
      mask Callback outputWidth: bus_expand_callback();
      mask Callback outputToWorkspace: bus_expand_callback();
  dout : Outport
  wires:
  reinterpret_out/1 -> dout/1
  din/1 -> reinterpret/1
  reinterpret/1 -> split/1(bus_in)
  join/1(bus_out) -> reinterpret_out/1
  split/1(msb_out9) -> join/1(in1), join/3(in3), join/5(in5), join/7(in7), join/9(in9), join/11(in11), join/13(in13), join/15(in15)
  split/9(lsb_out1) -> join/2(in2)
  split/8(out2) -> join/4(in4)
  split/7(out3) -> join/6(in6)
  split/6(out4) -> join/8(in8)
  split/5(out5) -> join/10(in10)
  split/4(out6) -> join/12(in12)
  split/3(out7) -> join/14(in14)
  split/2(out8) -> join/16(in16)

== system s_b16a4x512f/sys2/pkt_reord/munge1 ==
  din : Inport
  join : Subsystem  AncestorBlock=casper_library_flow_control/bus_create  mask(bus_create){inputNum=2}
      mask prompts: inputNum "Number of inputs:"
      mask init:
      | bus_create_init(gcb,...
      |     'inputNum', inputNum);
  reinterpret : xbsIndex_r4/Reinterpret  force_arith_type=on  arith_type=Unsigned  force_bin_pt=on  bin_pt=0  block_type=reinterpret
  reinterpret_out : xbsIndex_r4/Reinterpret  force_arith_type=on  arith_type=Unsigned  force_bin_pt=on  bin_pt=0  block_type=reinterpret
  split : Subsystem  AncestorBlock=casper_library_flow_control/bus_expand  mask(bus_expand){mode=divisions of arbitrary size, outputNum=1, outputWidth=[1 32], outputBinaryPt=[0 0], outputArithmeticType=[0 0], show_format=off, outputToWorkspace=off, variablePrefix=out, outputToModelAsWell=on}
      mask prompts: outputNum "Number of outputs:"; outputWidth "Output width [msb ... lsb]:"; outputBinaryPt "Output binary point position [msb ... lsb]:"; outputArithmeticType "Output arithmetic type (ufix=0, fix=1, bool=2) [msb ... lsb]:"; show_format "Print format string?"; outputToWorkspace "Output to workspace?"; variablePrefix "Variable name prefix:"; outputToModelAsWell "Output to model as well?"
      mask help:
      | Expands a 'bus' made using a bus_create or Xilinx
      | concat block.
      | The input will be divided into the specified number
      | of outputs with the specified arithmetic types.
      | Divisions are made from most significant bit.
      mask init: same as s_b16a4x512f/bus_expand
      settings: AttributesFormatString=2 outputs
      mask TypeOptions mode: divisions of equal size | divisions of arbitrary size
      mask Callback mode: bus_expand_callback();
      mask Callback outputWidth: bus_expand_callback();
      mask Callback outputToWorkspace: bus_expand_callback();
  dout : Outport
  wires:
  reinterpret_out/1 -> dout/1
  din/1 -> reinterpret/1
  reinterpret/1 -> split/1(bus_in)
  join/1(bus_out) -> reinterpret_out/1
  split/1(msb_out2) -> join/1(in1)
  split/2(lsb_out1) -> join/2(in2)

== system s_b16a4x512f/sys2/pkt_reord/output_control ==
  note: add delay here
      | to ensure mcnt has had
      | chance to calculate
      | correctly
  note: If reading from addr 0 (corresponding to f=0,nant,2nant,...)
      | and max_mcnt (skipping window_bits for the difference
      | between max_mcnt and rd_mcnt) is 0 for sync_bits, then
      | issue a sync.
  note: If we need to ship a window,
      | send the data on a window edge
  note: Decide whether to ship
      | a window or not:
  note: If the read window is 1/2
      | the total buffer size (or more)
      | behind the write window,
      | it is time to ship it out.
  note: rd_addr is counting for
      | output words to
      | X engines
  maxcnt : Inport
  AddSub1 : xbsIndex_r4/AddSub  mode=Subtraction  use_carryin=off  use_carryout=off  en=off  latency=2  precision=User Defined  arith_type=Unsigned  n_bits=window_bits  bin_pt=0  quantization=Truncate  overflow=Wrap  use_behavioral_HDL=on  hw_selection=Fabric  pipelined=off  use_rpm=on  dbl_ovrd=off  block_type=addsub
      settings: xl_area=[0, 0, 0, 0, 0, 0, 0]  block_version=10.1.3
  Concat1 : xbsIndex_r4/Concat  num_inputs=2  dbl_ovrd=off  block_type=concat
      settings: block_version=10.1.3
  Concat2 : xbsIndex_r4/Concat  num_inputs=2  dbl_ovrd=off  block_type=concat
      settings: block_version=10.1.3
  Constant1 : xbsIndex_r4/Constant  const=2^(window_bits - 1)  gui_display_data_type=Fixed-point  arith_type=Unsigned  n_bits=window_bits  bin_pt=0  preci_type=Single  exp_width=8  frac_width=24  explicit_period=on  period=1  equ=P=C  opselect=C  inp2=PCIN>>17  opr=+  inp1=P  carry=CIN  dbl_ovrd=off  block_type=constant
  Constant3 : xbsIndex_r4/Constant  const=0  gui_display_data_type=Fixed-point  arith_type=Unsigned  n_bits=sync_bits - x_int_bits - ant_bits - window_bits  bin_pt=0  preci_type=Single  exp_width=8  frac_width=24  explicit_period=on  period=1  equ=P=C  opselect=C  inp2=PCIN>>17  opr=+  inp1=P  carry=CIN  dbl_ovrd=off  block_type=constant
  Delay1 : xbsIndex_r4/Delay  rst=off  infoeditControl=Selection of Reset will increase slice count due to use of real FFs and instead of SRLs  en=off  latency=1  reg_retiming=on  dbl_ovrd=off  block_type=delay
      settings: xl_area=[0, 0, 0, 0, 0, 0, 0]
  Delay3 : xbsIndex_r4/Delay  rst=off  infoeditControl=Selection of Reset will increase slice count due to use of real FFs and instead of SRLs  en=off  latency=2  reg_retiming=on  dbl_ovrd=off  block_type=delay
      settings: xl_area=[0, 0, 0, 0, 0, 0, 0]
  Delay6 : xbsIndex_r4/Delay  rst=off  infoeditControl=Selection of Reset will increase slice count due to use of real FFs and instead of SRLs  en=off  latency=1  reg_retiming=on  dbl_ovrd=off  block_type=delay
      settings: xl_area=[0, 0, 0, 0, 0, 0, 0]
  Delay7 : xbsIndex_r4/Delay  rst=off  infoeditControl=Selection of Reset will increase slice count due to use of real FFs and instead of SRLs  en=off  latency=2  reg_retiming=on  dbl_ovrd=off  block_type=delay
      settings: xl_area=[0, 0, 0, 0, 0, 0, 0]
  Gateway Out{1..18} (18 alike) : xbsIndex_r4/Gateway Out  inherit_from_input=off  hdl_port=off  rows=1  columns=1  UseAsDAC=off  DACChannel='1'  interface=None  automatic_assignment=on  address_offset=hex2dec('00')  intf_name=''  intf_description=''  timing_constraint=None  locs_specified=off  LOCs={}  io_standard={}  block_type=gatewayout
      settings: infoedit="Gateway out block.  Converts Xilinx fixed point inputs into ouputs of type Simulink integer, double, or fixed point.<P><P>Hardware notes:  In hardware these blocks become top level output ports or are discarded, depending on how they are configured."  xl_area=[0, 0, 0, 0, 0, 0, 0]  block_version=10.1.3
  Logical1 : xbsIndex_r4/Logical  logical_function=AND  inputs=2  en=off  latency=0  precision=Full  arith_type=Unsigned  n_bits=8  bin_pt=2  align_bp=on  dbl_ovrd=off  block_type=logical
      settings: xl_area=[0, 0, 0, 0, 0, 0, 0]
  Logical2 : xbsIndex_r4/Logical  logical_function=AND  inputs=2  en=off  latency=0  precision=Full  arith_type=Unsigned  n_bits=8  bin_pt=2  align_bp=on  dbl_ovrd=off  block_type=logical
      settings: xl_area=[0, 0, 0, 0, 0, 0, 0]
  Logical4 : xbsIndex_r4/Logical  logical_function=AND  inputs=2  en=off  latency=0  precision=Full  arith_type=Unsigned  n_bits=8  bin_pt=2  align_bp=on  dbl_ovrd=off  block_type=logical
      settings: xl_area=[0, 0, 0, 0, 0, 0, 0]
  Register : xbsIndex_r4/Register  init=0  rst=off  en=on  dbl_ovrd=off  block_type=register
  Register1 : xbsIndex_r4/Register  init=0  rst=off  en=on  dbl_ovrd=off  block_type=register
  Register3 : xbsIndex_r4/Register  init=0  rst=off  en=on  dbl_ovrd=off  block_type=register
  Relational1 : xbsIndex_r4/Relational  mode=a>=b  op_type=Bool  en=off  latency=1  dbl_ovrd=off  block_type=relational
      settings: xl_area=[0, 0, 0, 0, 0, 0, 0]  block_version=10.1.3
  Relational4 : xbsIndex_r4/Relational  mode=a=b  op_type=Bool  en=off  latency=1  dbl_ovrd=off  block_type=relational
      settings: xl_area=[0, 0, 0, 0, 0, 0, 0]  block_version=10.1.3
  Slice1 : xbsIndex_r4/Slice  nbits=window_bits  boolean_output=off  mode=Lower Bit Location + Width  bit1=0  base1=MSB of Input  bit0=0  base0=LSB of Input  dbl_ovrd=off  block_type=slice
      settings: infoedit="Extracts a given range of bits from each input sample and presents it at the output.  The output type is ordinarily unsigned with binary point at zero, but can be Boolean when the slice is one bit wide.<P><P>Hardware notes: In hardware this block costs nothing."  block_version=10.1.3
  Slice2 : xbsIndex_r4/Slice  nbits=1  boolean_output=on  mode=Upper Bit Location + Width  bit1=0  base1=MSB of Input  bit0=0  base0=LSB of Input  dbl_ovrd=off  block_type=slice
      settings: infoedit="Extracts a given range of bits from each input sample and presents it at the output.  The output type is ordinarily unsigned with binary point at zero, but can be Boolean when the slice is one bit wide.<P><P>Hardware notes: In hardware this block costs nothing."  block_version=10.1.3
  Slice3 : xbsIndex_r4/Slice  nbits=window_bits  boolean_output=off  mode=Lower Bit Location + Width  bit1=0  base1=MSB of Input  bit0=0  base0=LSB of Input  dbl_ovrd=off  block_type=slice
      settings: infoedit="Extracts a given range of bits from each input sample and presents it at the output.  The output type is ordinarily unsigned with binary point at zero, but can be Boolean when the slice is one bit wide.<P><P>Hardware notes: In hardware this block costs nothing."  block_version=10.1.3
  Slice4 : xbsIndex_r4/Slice  nbits=x_int_bits + ant_bits - n_bits_output_words  boolean_output=off  mode=Lower Bit Location + Width  bit1=0  base1=MSB of Input  bit0=0  base0=LSB of Input  dbl_ovrd=off  block_type=slice
      settings: block_version=10.1.3
  Slice5 : xbsIndex_r4/Slice  nbits=window_bits  boolean_output=off  mode=Two Bit Locations  bit1=sync_bits - x_int_bits - ant_bits - 1  base1=LSB of Input  bit0=window_bits  base0=LSB of Input  dbl_ovrd=off  block_type=slice
      settings: infoedit="Extracts a given range of bits from each input sample and presents it at the output.  The output type is ordinarily unsigned with binary point at zero, but can be Boolean when the slice is one bit wide.<P><P>Hardware notes: In hardware this block costs nothing."  block_version=10.1.3
  Slice6 : xbsIndex_r4/Slice  nbits=1  boolean_output=on  mode=Upper Bit Location + Width  bit1=0  base1=MSB of Input  bit0=0  base0=LSB of Input  dbl_ovrd=off  block_type=slice
      settings: infoedit="Extracts a given range of bits from each input sample and presents it at the output.  The output type is ordinarily unsigned with binary point at zero, but can be Boolean when the slice is one bit wide.<P><P>Hardware notes: In hardware this block costs nothing."  block_version=10.1.3
  Slice7 : xbsIndex_r4/Slice  nbits=1  boolean_output=off  mode=Two Bit Locations  bit1=0  base1=MSB of Input  bit0=window_bits  base0=LSB of Input  dbl_ovrd=off  block_type=slice
      settings: infoedit="Extracts a given range of bits from each input sample and presents it at the output.  The output type is ordinarily unsigned with binary point at zero, but can be Boolean when the slice is one bit wide.<P><P>Hardware notes: In hardware this block costs nothing."  block_version=10.1.3
  edge_detect : Subsystem  AncestorBlock=casper_library_misc/edge_detect  mask(edge_detect){edge=Both, polarity=Active High, x_in=[0 0.08 0.08 0.16 0.16 0.24 0.24 0.32 0.32 0.4], y_in=[-1 -1  1  1  1  1  1  1  1  1], x_out=[0.6 0.68 0.68 0.76 0.76 0.84 0.84 0.92 0.92 1], y_out=[-1 -1  1  1 -1 -1 -1 -1 -1 -1]}
      mask prompts: edge "Edge Type"; polarity "Output Polarity"; x_in "Input X Positions"; y_in "Input Y Positions"; x_out "Output X Positions"; y_out "Output Y Positions"
      mask help: Output is active for one-cycle after each edge of the specified type (i.e. rising, falling or both).
      mask init: same as s_b16a4x512f/edge_detect
      settings: AttributesFormatString=|
      | both edges
      | active high
      mask Help: Output is active for one-cycle after each edge of the specified type (i.e. rising, falling, or both).  Latency is zero.
      mask TypeOptions edge: Rising | Falling | Both
      mask TypeOptions polarity: Active High | Active Low
      mask Display:
      | plot(x_in_num,0.5+y_in_num*0.2);
      | plot(x_out_num,0.5+y_out_num*0.2);
  edge_detect1 : Subsystem  AncestorBlock=casper_library_misc/edge_detect  mask(edge_detect){edge=Both, polarity=Active High, x_in=[0 0.08 0.08 0.16 0.16 0.24 0.24 0.32 0.32 0.4], y_in=[-1 -1  1  1  1  1  1  1  1  1], x_out=[0.6 0.68 0.68 0.76 0.76 0.84 0.84 0.92 0.92 1], y_out=[-1 -1  1  1 -1 -1 -1 -1 -1 -1]}
      mask prompts: edge "Edge Type"; polarity "Output Polarity"; x_in "Input X Positions"; y_in "Input Y Positions"; x_out "Output X Positions"; y_out "Output Y Positions"
      mask help: Output is active for one-cycle after each edge of the specified type (i.e. rising, falling or both).
      mask init: same as s_b16a4x512f/edge_detect
      settings: AttributesFormatString=|
      | both edges
      | active high
      mask Help: Output is active for one-cycle after each edge of the specified type (i.e. rising, falling, or both).  Latency is zero.
      mask TypeOptions edge: Rising | Falling | Both
      mask TypeOptions polarity: Active High | Active Low
      mask Display:
      | plot(x_in_num,0.5+y_in_num*0.2);
      | plot(x_out_num,0.5+y_out_num*0.2);
  internal_descr_Scope : Scope  NumInputPorts=8
  internal_descr_Scope1 : Scope  NumInputPorts=10
  pulse_ext : Subsystem  AncestorBlock=casper_library/Misc/pulse_ext  mask(pulse_ext){pulse_len=2^(x_int_bits + ant_bits - n_bits_output_words)}
      mask prompts: pulse_len "Length of Pulse"
      mask help:
      | Extends a boolean signal to be high for the specified number of clocks after
      | the last high input.
      mask init:
      | bits = ceil(log2(pulse_len+1));
      mask Help: eval('xlWeb([getenv(''MLIB_ROOT''), ''\doc\htmlblocks\sp_pulse_ext\sp_pulse_ext.html''])')
  win_addr_cnt : xbsIndex_r4/Counter  cnt_type=Free Running  cnt_to=Inf  operation=Up  start_count=0  cnt_by_val=1  arith_type=Unsigned  n_bits=x_int_bits + ant_bits + 1 - n_bits_output_words  bin_pt=0  load_pin=off  rst=off  en=off  explicit_period=on  period=1  use_behavioral_HDL=off  implementation=Fabric  use_rpm=on  dbl_ovrd=off  block_type=counter
      settings: xl_area=[0, 0, 0, 0, 0, 0, 0]
  win_cnt : xbsIndex_r4/Counter  cnt_type=Free Running  cnt_to=Inf  operation=Up  start_count=0  cnt_by_val=1  arith_type=Unsigned  n_bits=window_bits + 1  bin_pt=0  load_pin=off  rst=off  en=on  explicit_period=off  period=1  use_behavioral_HDL=off  implementation=Fabric  use_rpm=on  dbl_ovrd=off  block_type=counter
      settings: xl_area=[0, 0, 0, 0, 0, 0, 0]
  gen_sync : Outport
  rd_en : Outport  Port=2
  rd_addr : Outport  Port=3
  rd_timefreq : Outport  Port=4
  wires:
  [current_window_out] -> Concat1/1
  [buffer_edge] -> [mcnt_sample], Register/2
  Gateway Out18/1 -> internal_descr_Scope1/10
  [sampled_mcnt] -> Gateway Out18/1
  Register/1 -> Concat2/1, [sampled_mcnt]
  Slice7/1 -> Register/1
  [maxcnt] -> Slice7/1, [offset_mcnt]
  Delay3/1 -> Logical1/2
  Gateway Out17/1 -> internal_descr_Scope1/9
  [mcnt_sample] -> Gateway Out17/1
  [rd_addr] -> Gateway Out2/1
  [rd_en] -> Gateway Out1/1
  [rd_addr] -> Gateway Out14/1
  [rd_en] -> Gateway Out9/1
  [rd_mcnt] -> Gateway Out13/1
  [ship_next_window] -> Gateway Out8/1
  [offset_mcnt] -> Gateway Out12/1
  [maxcnt] -> Gateway Out10/1
  [current_window_out] -> Gateway Out11/1
  Delay1/1 -> [current_window_out]
  win_cnt/1 -> Register1/1
  Delay6/1 -> Logical4/1
  Register3/1 -> Logical4/2
  pulse_ext/1(out) -> Delay6/1
  Logical4/1 -> [rd_en], rd_en/1
  [rd_mcnt] -> Gateway Out7/1
  Logical2/1 -> [gen_sync], gen_sync/1
  Gateway Out16/1 -> internal_descr_Scope/8
  [gen_sync] -> Gateway Out16/1
  [gen_sync] -> Gateway Out15/1
  Gateway Out15/1 -> internal_descr_Scope1/8
  Gateway Out14/1 -> internal_descr_Scope1/7
  Gateway Out9/1 -> internal_descr_Scope1/6
  Gateway Out8/1 -> internal_descr_Scope1/5
  Gateway Out13/1 -> internal_descr_Scope1/4
  Gateway Out12/1 -> internal_descr_Scope1/3
  Gateway Out11/1 -> internal_descr_Scope1/1
  Gateway Out10/1 -> internal_descr_Scope1/2
  [current_window_out] -> Concat2/2
  Gateway Out7/1 -> internal_descr_Scope/7
  [ship_window_now] -> Gateway Out6/1
  Gateway Out2/1 -> internal_descr_Scope/6
  Gateway Out1/1 -> internal_descr_Scope/5
  Gateway Out6/1 -> internal_descr_Scope/4
  [ship_next_window] -> Gateway Out5/1
  [current_window_out] -> Gateway Out3/1
  [maxcnt] -> Gateway Out4/1
  Gateway Out5/1 -> internal_descr_Scope/3
  Gateway Out4/1 -> internal_descr_Scope/1
  Gateway Out3/1 -> internal_descr_Scope/2
  Relational4/1 -> Logical2/2
  [ship_window_now] -> Register1/2, win_cnt/1
  Relational1/1 -> [ship_next_window]
  [maxcnt] -> Slice3/1
  [current_window] -> AddSub1/2
  Constant1/1 -> Relational1/2
  AddSub1/1 -> Relational1/1
  Slice3/1 -> AddSub1/1
  [ship_next_window] -> Delay3/1
  maxcnt/1 -> Slice5/1, [maxcnt]
  Register1/1 -> Slice2/1, Slice1/1
  Logical1/1 -> [ship_window_now], pulse_ext/1(in), Register3/2, Register3/1
  edge_detect/1(out) -> [buffer_edge], Logical2/1
  Constant3/1 -> Relational4/1
  Slice5/1 -> Relational4/2
  win_addr_cnt/1 -> Slice6/1, Slice4/1
  Slice6/1 -> edge_detect1/1(in)
  edge_detect1/1(out) -> Logical1/1
  Slice4/1 -> Delay7/1
  Slice1/1 -> Delay1/1, [current_window]
  Slice2/1 -> edge_detect/1(in)
  Delay7/1 -> Concat1/2
  Concat1/1 -> [rd_addr], rd_addr/1
  Concat2/1 -> rd_timefreq/1, [rd_mcnt]

== system s_b16a4x512f/sys2/pkt_reord/time_freq_unpack ==
  din : Inport
  xeng_id : Inport  Port=2
  Concat2 : xbsIndex_r4/Concat  num_inputs=2  dbl_ovrd=off  block_type=concat
  Slice2 : xbsIndex_r4/Slice  nbits=chan_bits-xeng_bits  boolean_output=off  mode=Lower Bit Location + Width  bit1=-1  base1=MSB of Input  bit0=0  base0=LSB of Input  dbl_ovrd=off  block_type=slice
      settings: block_version=10.1.3
  Slice3 : xbsIndex_r4/Slice  nbits=1  boolean_output=off  mode=Two Bit Locations  bit1=0  base1=MSB of Input  bit0=chan_bits-xeng_bits  base0=LSB of Input  dbl_ovrd=off  block_type=slice
      settings: block_version=10.1.3
  time : Outport
  freq : Outport  Port=2
  wires:
  xeng_id/1 -> Concat2/1
  Concat2/1 -> freq/1
  Slice2/1 -> Concat2/2
  Slice3/1 -> time/1
  din/1 -> Slice2/1, Slice3/1
